simulink model "Test01_SIG_Ctrl_2019a"  (R2019a)
settings: Solver=ode4  StartTime=0.0  StopTime=TMax  FixedStep=DT  MaxStep=DT  RelTol=1e-3  EnableMultiTasking=on
values from neighbouring files (symbols this model uses):
  a0 = -wecs.Bt/wecs.mt    [calcDiscretParamTowerMotion.m]
  a1 = -wecs.Kt/wecs.mt    [calcDiscretParamTowerMotion.m]
  c1 = fmtCell(data{r}(1), nf, doNorm)    [merge_stats_tables_norm.m]
  c2 = fmtCell(data{r}(2), nf, doNorm)    [merge_stats_tables_norm.m]
  IPC_KI_1p = xCtrl(1)    [runSimIPC.m]
  IPC_KP_1p = xCtrl(2)    [runSimIPC.m]
  kp_Turm = xCtrl(3)    [runSimIPC.m]
  OutList = OutTable.Properties.VariableNames    [initLPVParam.m]    (also in testCtrl.m; testOutList.m = cell(40, 1); testqLPV.m = cell(40, 1))
undefined symbols (not defined in the file or in its folder): b0, b0Torque, b1, b1Torque, d1, d2, d3, GBoxEff, GBRatio, GK_Start, IPC_An, IPC_K_1P, k_Pitch, M_Gen_change_max, M_Gen_max, M_Gen_min, MaxPit, MinPit, offest_1p, PC_KI, PC_KK, PC_KP, Pitch_change_max, RPM_Init, strmatch, switchOrigFiltGenSpeed, T_Turmfilter, v_Gen_nenn
libraries: simulink x4, simulink_extras x2
settings Model: Creator=bjonkman  LastModifiedBy=ditt_aj
settings DataIOCC: SaveFormat=Array  SignalLoggingSaveFormat=ModelDataLogs  SaveOutput=off  SaveTime=off  ReturnWorkspaceOutputs=off  SignalLoggingName=sigsOut
settings OptimizationCC: ExpressionDepthLimit=2147483647  LifeSpan=inf
settings DebuggingCC: SaveWithParameterizedLinksMsg=none  UnderspecifiedInitializationDetection=Classic  MergeDetectMultiDrivingBlocksExec=none  SignalResolutionControl=TryResolveAllWithWarning  MultiTaskDSMMsg=warning  MultiTaskCondExecSysMsg=none  FcnCallInpInsideContextMsg=warning  StateNameClashWarn=warning  SFUnexpectedBacktrackingDiag=warning  SFNoUnconditionalDefaultTransitionDiag=warning  ArithmeticOperatorsInVariantConditions=warning
settings HardwareCC: ProdBitPerPointer=32  ProdBitPerSizeT=32  ProdBitPerPtrDiffT=32  ProdLargestAtomicFloat=None  ProdIntDivRoundTo=Undefined  ProdEndianess=Unspecified  ProdWordSize=32  ProdHWDeviceType=32-bit Generic  TargetUnknown=on
settings ModelReferenceCC: PropagateSignalLabelsOutOfModel=off
settings SFSimCC: SimUseLocalCustomCode=off
settings RTWCC: RTWUseLocalCustomCode=off
settings CodeAppCC: StateflowObjectComments=on
settings GRTTargetCC: TargetLangStandard=C89/C90 (ANSI)  ModelReferenceCompliant=off  ParMdlRefBuildCompliant=off  CompOptLevelCompliant=off  ConcurrentExecutionCompliant=off  GeneratePreprocessorConditionals=Disable all  CombineOutputUpdateFcns=off  MatFileLogging=off  GRTInterface=on
settings ConfigComp: CovMetricSettings=dw  CovHtmlReporting=on  CovSaveCumulativeToWorkspaceVar=on  CovSaveSingleToWorkspaceVar=on  CovExternalEMLEnable=off

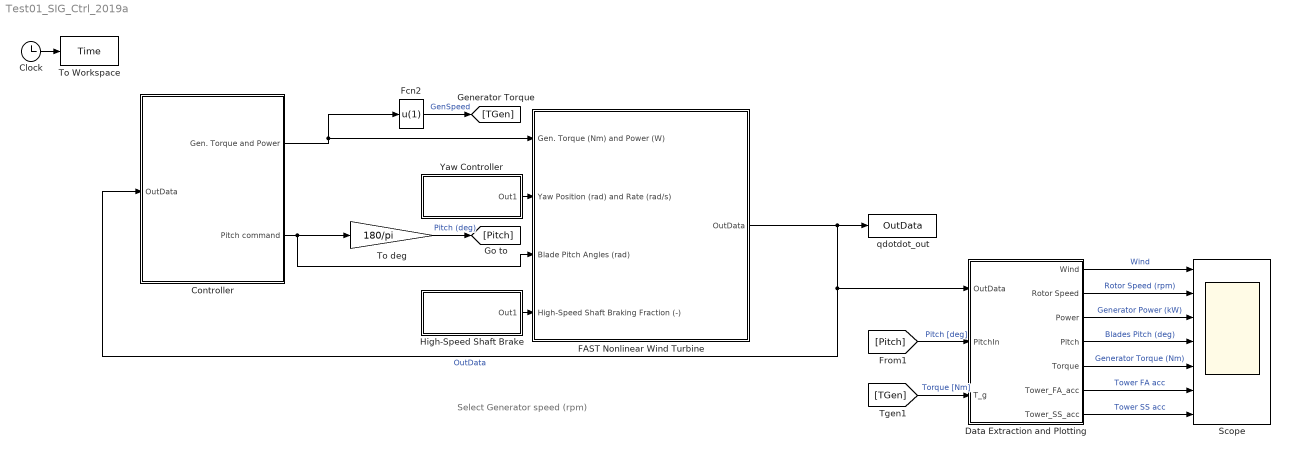
== system Test01_SIG_Ctrl_2019a ==
  note: Select Generator speed (rpm)
  Clock : Clock
  Controller : Subsystem
  Data Extraction and Plotting : Subsystem
  FAST Nonlinear Wind Turbine : Subsystem  mask(FAST Nonlinear Wind Turbine){}
      mask help: This block contains the FAST S-Function.
      mask init:
      | clear FAST_SFunc
  Fcn2 : Fcn  Expr=u(1)
  High-Speed Shaft Brake : Subsystem
  Scope : Scope  NumInputPorts=7
      settings: Tag=Scope
  To Workspace : ToWorkspace  VariableName=Time  SampleTime=-1
  To deg : Gain  Gain=180/pi
  Yaw Controller : Subsystem
  qdotdot_out : ToWorkspace  VariableName=OutData  SampleTime=-1
  wires:
  Clock/1 -> To Workspace/1
  Yaw Controller/1(Out1) -> FAST Nonlinear Wind Turbine/2(Yaw Position (rad) and Rate (rad/s))
  High-Speed Shaft Brake/1(Out1) -> FAST Nonlinear Wind Turbine/4(High-Speed Shaft Braking Fraction (-))
  FAST Nonlinear Wind Turbine/1(OutData) -> qdotdot_out/1, Data Extraction and Plotting/1(OutData), Controller/1(OutData)  "OutData"
  Fcn2/1 -> [TGen]  "GenSpeed"
  Data Extraction and Plotting/2(Rotor Speed) -> Scope/2  "Rotor Speed (rpm)"
  Data Extraction and Plotting/4(Pitch) -> Scope/4  "Blades Pitch (deg)"
  Data Extraction and Plotting/3(Power) -> Scope/3  "Generator Power (kW)"
  [TGen] -> Data Extraction and Plotting/3(T_g)  "Torque [Nm]"
  Data Extraction and Plotting/5(Torque) -> Scope/5  "Generator Torque (Nm)"
  [Pitch] -> Data Extraction and Plotting/2(PitchIn)  "Pitch [deg]"
  Data Extraction and Plotting/7(Tower_SS_acc) -> Scope/7  "Tower SS acc"
  Data Extraction and Plotting/6(Tower_FA_acc) -> Scope/6  "Tower FA acc"
  Data Extraction and Plotting/1(Wind) -> Scope/1  "Wind"
  To deg/1 -> [Pitch]  "Pitch (deg)"
  Controller/2(Pitch command) -> FAST Nonlinear Wind Turbine/3(Blade Pitch Angles (rad)), To deg/1
  Controller/1(Gen. Torque and Power) -> FAST Nonlinear Wind Turbine/1(Gen. Torque (Nm) and Power (W)), Fcn2/1

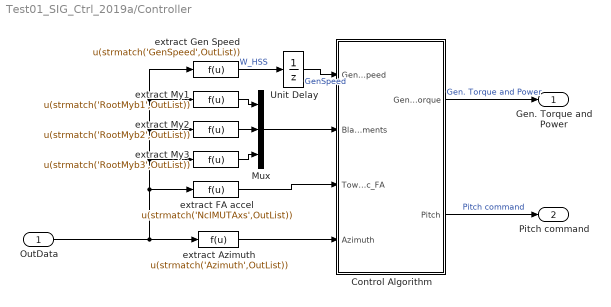
== system Test01_SIG_Ctrl_2019a/Controller ==
  OutData : Inport
  Control Algorithm : Subsystem
  Mux : Mux  Inputs=3
  Unit Delay : UnitDelay  InitialCondition=RPM_Init*GBRatio  SampleTime=-1  HasFrameUpgradeWarning=on
  extract Azimuth : Fcn  Expr=u(strmatch('Azimuth',OutList))
  extract FA accel : Fcn  Expr=u(strmatch('NcIMUTAxs',OutList))
  extract Gen Speed : Fcn  Expr=u(strmatch('GenSpeed',OutList))
  extract My1 : Fcn  Expr=u(strmatch('RootMyb1',OutList))
  extract My2 : Fcn  Expr=u(strmatch('RootMyb2',OutList))
  extract My3 : Fcn  Expr=u(strmatch('RootMyb3',OutList))
  Gen. Torque and Power : Outport
  Pitch command : Outport  Port=2
  wires:
  extract Azimuth/1 -> Control Algorithm/4(Azimuth)
  OutData/1 -> extract Gen Speed/1, extract My1/1, extract My2/1, extract My3/1, extract FA accel/1, extract Azimuth/1
  Unit Delay/1 -> Control Algorithm/1(Generator_Speed)  "GenSpeed"
  extract My3/1 -> Mux/3
  extract FA accel/1 -> Control Algorithm/3(TowerAcc_FA)
  extract My2/1 -> Mux/2
  extract My1/1 -> Mux/1
  Mux/1 -> Control Algorithm/2(Blade_Moments)
  extract Gen Speed/1 -> Unit Delay/1  "W_HSS"
  Control Algorithm/1(Generator_Torque) -> Gen. Torque and Power/1  "Gen. Torque and Power"
  Control Algorithm/2(Pitch) -> Pitch command/1  "Pitch command"

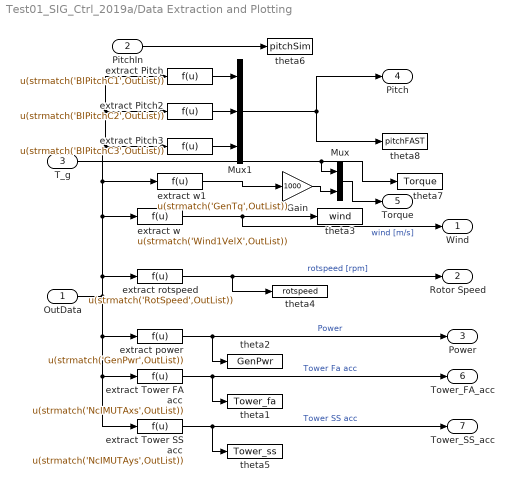
== system Test01_SIG_Ctrl_2019a/Data Extraction and Plotting ==
  OutData : Inport
  PitchIn : Inport  Port=2
  T_g : Inport  Port=3
  Gain : Gain  Gain=1000
  Mux : Mux  Inputs=2
  Mux1 : Mux  Inputs=3
  extract Pitch : Fcn  Expr=u(strmatch('BlPitchC1',OutList))
  extract Pitch2 : Fcn  Expr=u(strmatch('BlPitchC2',OutList))
  extract Pitch3 : Fcn  Expr=u(strmatch('BlPitchC3',OutList))
  extract Tower FA acc : Fcn  Expr=u(strmatch('NcIMUTAxs',OutList))
  extract Tower SS acc : Fcn  Expr=u(strmatch('NcIMUTAys',OutList))
  extract power : Fcn  Expr=u(strmatch('GenPwr',OutList))
  extract rotspeed : Fcn  Expr=u(strmatch('RotSpeed',OutList))
  extract w : Fcn  Expr=u(strmatch('Wind1VelX',OutList))
  extract w1 : Fcn  Expr=u(strmatch('GenTq',OutList))
  theta1 : ToWorkspace  VariableName=Tower_fa  SampleTime=-1
      settings: MaxDataPoints=Inf  Decimation=3
  theta2 : ToWorkspace  VariableName=GenPwr  SampleTime=-1
      settings: MaxDataPoints=Inf  Decimation=3
  theta3 : ToWorkspace  VariableName=wind  SampleTime=-1
      settings: MaxDataPoints=Inf  Decimation=3
  theta4 : ToWorkspace  VariableName=rotspeed  SampleTime=-1
      settings: MaxDataPoints=Inf  Decimation=3
  theta5 : ToWorkspace  VariableName=Tower_ss  SampleTime=-1
      settings: MaxDataPoints=Inf  Decimation=3
  theta6 : ToWorkspace  VariableName=pitchSim  SampleTime=-1
      settings: MaxDataPoints=Inf  Decimation=3
  theta7 : ToWorkspace  VariableName=Torque  SampleTime=-1
      settings: MaxDataPoints=Inf  Decimation=3
  theta8 : ToWorkspace  VariableName=pitchFAST  SampleTime=-1
      settings: MaxDataPoints=Inf  Decimation=3
  Wind : Outport
  Rotor Speed : Outport  Port=2
  Power : Outport  Port=3
  Pitch : Outport  Port=4
  Torque : Outport  Port=5
  Tower_FA_acc : Outport  Port=6
  Tower_SS_acc : Outport  Port=7
  wires:
  extract w/1 -> Wind/1, theta3/1  "wind [m/s]"
  extract rotspeed/1 -> theta4/1, Rotor Speed/1  "rotspeed [rpm]"
  extract power/1 -> theta2/1, Power/1  "Power"
  T_g/1 -> Mux/1, theta7/1
  extract Tower FA acc/1 -> theta1/1, Tower_FA_acc/1  "Tower Fa acc"
  OutData/1 -> extract w/1, extract Pitch/1, extract Pitch2/1, extract Pitch3/1, extract w1/1, extract rotspeed/1, extract Tower SS acc/1, extract Tower FA acc/1, extract power/1
  extract Tower SS acc/1 -> theta5/1, Tower_SS_acc/1  "Tower SS acc"
  extract w1/1 -> Gain/1
  Gain/1 -> Mux/2
  Mux/1 -> Torque/1
  PitchIn/1 -> theta6/1
  Mux1/1 -> theta8/1, Pitch/1
  extract Pitch3/1 -> Mux1/3
  extract Pitch/1 -> Mux1/1
  extract Pitch2/1 -> Mux1/2

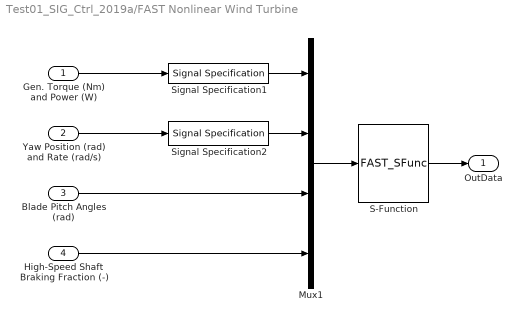
== system Test01_SIG_Ctrl_2019a/FAST Nonlinear Wind Turbine ==
  Gen. Torque (Nm) and Power (W) : Inport
  Yaw Position (rad) and Rate (rad/s) : Inport  Port=2
  Blade Pitch Angles (rad) : Inport  Port=3
  High-Speed Shaft Braking Fraction (-) : Inport  Port=4
  Mux1 : Mux
  S-Function : S-Function  FunctionName=FAST_SFunc  Parameters=FAST_InputFileName, TMax, 0  SFunctionDeploymentMode=off  EnableBusSupport=off
  Signal Specification1 : SignalSpecification  OutDataTypeStr=double  Dimensions=2
  Signal Specification2 : SignalSpecification  OutDataTypeStr=double  Dimensions=2
  OutData : Outport
  wires:
  Gen. Torque (Nm) and Power (W)/1 -> Signal Specification1/1
  S-Function/1 -> OutData/1
  Mux1/1 -> S-Function/1
  Blade Pitch Angles (rad)/1 -> Mux1/3
  Yaw Position (rad) and Rate (rad/s)/1 -> Signal Specification2/1
  Signal Specification1/1 -> Mux1/1
  Signal Specification2/1 -> Mux1/2
  High-Speed Shaft Braking Fraction (-)/1 -> Mux1/4

== system Test01_SIG_Ctrl_2019a/High-Speed Shaft Brake ==
  High-Speed Shaft Braking Fraction : Constant  Value=0
  Out1 : Outport
  wires:
  High-Speed Shaft Braking Fraction/1 -> Out1/1

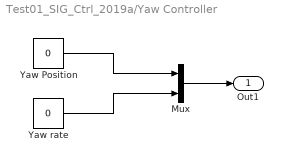
== system Test01_SIG_Ctrl_2019a/Yaw Controller ==
  Mux : Mux  Inputs=2
  Yaw Position : Constant  Value=0
  Yaw rate : Constant  Value=0
  Out1 : Outport
  wires:
  Mux/1 -> Out1/1
  Yaw Position/1 -> Mux/1
  Yaw rate/1 -> Mux/2

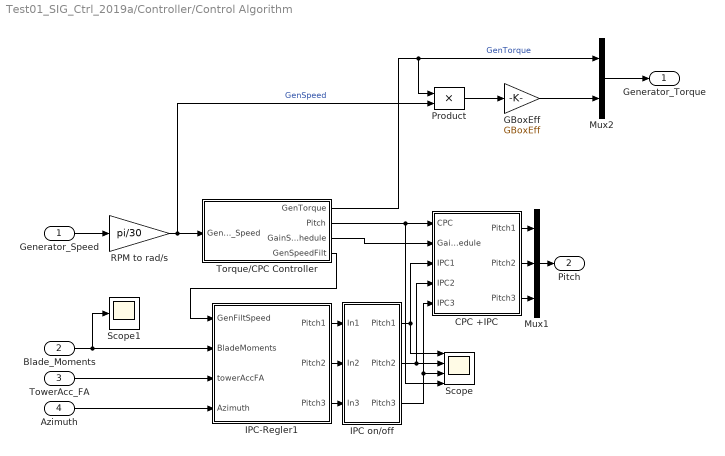
== system Test01_SIG_Ctrl_2019a/Controller/Control Algorithm ==
  Generator_Speed : Inport
  Blade_Moments : Inport  Port=2
  TowerAcc_FA : Inport  Port=3
  Azimuth : Inport  Port=4
  CPC +IPC : Subsystem
  GBoxEff : Gain  Gain=GBoxEff
  IPC on/off : Subsystem
  IPC-Regler1 : Subsystem
  Mux1 : Mux  Inputs=3
  Mux2 : Mux  Inputs=2
  Product : Product  RndMeth=Zero
  RPM to rad/s : Gain  Gain=pi/30  SaturateOnIntegerOverflow=on  OutDataTypeStr=Inherit: Same as input  ParamDataTypeStr=Inherit: Same as input
  Scope : Scope  NumInputPorts=4
  Scope1 : Scope
  Torque/CPC Controller : Subsystem
  Generator_Torque : Outport
  Pitch : Outport  Port=2
  wires:
  IPC on/off/3(Pitch3) -> CPC +IPC/5(IPC3), Scope/3
  Torque/CPC Controller/4(GenSpeedFilt) -> IPC-Regler1/1(GenFiltSpeed)
  IPC on/off/1(Pitch1) -> CPC +IPC/3(IPC1), Scope/1
  Torque/CPC Controller/2(Pitch) -> Scope/4, CPC +IPC/1(CPC)
  CPC +IPC/3(Pitch3) -> Mux1/3
  IPC on/off/2(Pitch2) -> CPC +IPC/4(IPC2), Scope/2
  IPC-Regler1/3(Pitch3) -> IPC on/off/3(In3)
  IPC-Regler1/1(Pitch1) -> IPC on/off/1(In1)
  IPC-Regler1/2(Pitch2) -> IPC on/off/2(In2)
  Torque/CPC Controller/3(GainSchedule) -> CPC +IPC/2(GainSchedule)
  CPC +IPC/1(Pitch1) -> Mux1/1
  CPC +IPC/2(Pitch2) -> Mux1/2
  Azimuth/1 -> IPC-Regler1/4(Azimuth)
  Torque/CPC Controller/1(GenTorque) -> Mux2/1, Product/1  "GenTorque"
  Blade_Moments/1 -> Scope1/1, IPC-Regler1/2(BladeMoments)
  Mux1/1 -> Pitch/1
  TowerAcc_FA/1 -> IPC-Regler1/3(towerAccFA)
  Product/1 -> GBoxEff/1
  Generator_Speed/1 -> RPM to rad/s/1
  GBoxEff/1 -> Mux2/2
  Mux2/1 -> Generator_Torque/1
  RPM to rad/s/1 -> Product/2, Torque/CPC Controller/1(Generator_Speed)  "GenSpeed"

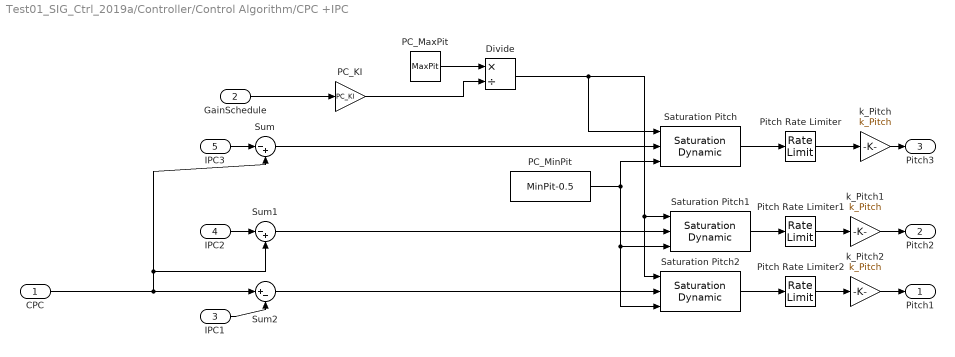
== system Test01_SIG_Ctrl_2019a/Controller/Control Algorithm/CPC +IPC ==
  CPC : Inport
  GainSchedule : Inport  Port=2
  IPC1 : Inport  Port=3
  IPC2 : Inport  Port=4
  IPC3 : Inport  Port=5
  Divide : Product  Inputs=*/
  PC_KI : Gain  Gain=PC_KI
  PC_MaxPit : Constant  Value=MaxPit
  PC_MinPit : Constant  Value=MinPit-0.5
  Pitch Rate Limiter : RateLimiter  RisingSlewLimit=Pitch_change_max  FallingSlewLimit=-Pitch_change_max  SampleTimeMode=inherited
  Pitch Rate Limiter1 : RateLimiter  RisingSlewLimit=Pitch_change_max  FallingSlewLimit=-Pitch_change_max  SampleTimeMode=inherited
  Pitch Rate Limiter2 : RateLimiter  RisingSlewLimit=Pitch_change_max  FallingSlewLimit=-Pitch_change_max  SampleTimeMode=inherited
  Saturation Pitch : simulink/Discontinuities/Saturation Dynamic  OutMin=[]  OutMax=[]  OutDataTypeStr=Inherit: Same as second input  OutDataType=fixdt(1, 16)  OutScaling=2^-10  DoSatur=off
  Saturation Pitch1 : simulink/Discontinuities/Saturation Dynamic  OutMin=[]  OutMax=[]  OutDataTypeStr=Inherit: Same as second input  OutDataType=fixdt(1, 16)  OutScaling=2^-10  DoSatur=off
  Saturation Pitch2 : simulink/Discontinuities/Saturation Dynamic  OutMin=[]  OutMax=[]  OutDataTypeStr=Inherit: Same as second input  OutDataType=fixdt(1, 16)  OutScaling=2^-10  DoSatur=off
  Sum : Sum  Inputs=|-+
  Sum1 : Sum  Inputs=|-+
  Sum2 : Sum  Inputs=|+-
  k_Pitch : Gain  Gain=k_Pitch
  k_Pitch1 : Gain  Gain=k_Pitch
  k_Pitch2 : Gain  Gain=k_Pitch
  Pitch1 : Outport
  Pitch2 : Outport  Port=2
  Pitch3 : Outport  Port=3
  wires:
  PC_KI/1 -> Divide/2
  PC_MinPit/1 -> Saturation Pitch1/3, Saturation Pitch2/3, Saturation Pitch/3
  Saturation Pitch/1 -> Pitch Rate Limiter/1
  Pitch Rate Limiter1/1 -> k_Pitch1/1
  Divide/1 -> Saturation Pitch1/1, Saturation Pitch2/1, Saturation Pitch/1
  Pitch Rate Limiter2/1 -> k_Pitch2/1
  Pitch Rate Limiter/1 -> k_Pitch/1
  Sum1/1 -> Saturation Pitch1/2
  PC_MaxPit/1 -> Divide/1
  Sum2/1 -> Saturation Pitch2/2
  IPC3/1 -> Sum/1
  Saturation Pitch1/1 -> Pitch Rate Limiter1/1
  k_Pitch1/1 -> Pitch2/1
  Sum/1 -> Saturation Pitch/2
  Saturation Pitch2/1 -> Pitch Rate Limiter2/1
  IPC2/1 -> Sum1/1
  k_Pitch/1 -> Pitch3/1
  GainSchedule/1 -> PC_KI/1
  IPC1/1 -> Sum2/2
  CPC/1 -> Sum1/2, Sum/2, Sum2/1
  k_Pitch2/1 -> Pitch1/1

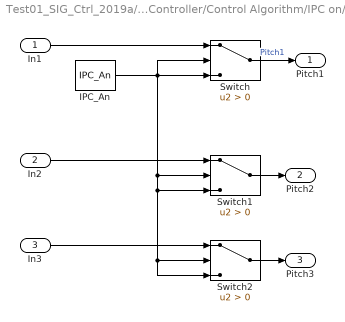
== system Test01_SIG_Ctrl_2019a/Controller/Control Algorithm/IPC on//off ==
  In1 : Inport
  In2 : Inport  Port=2
  In3 : Inport  Port=3
  IPC_An : Constant  Value=IPC_An
  Switch : Switch  Criteria=u2 > Threshold
  Switch1 : Switch  Criteria=u2 > Threshold
  Switch2 : Switch  Criteria=u2 > Threshold
  Pitch1 : Outport
  Pitch2 : Outport  Port=2
  Pitch3 : Outport  Port=3
  wires:
  Switch1/1 -> Pitch2/1
  IPC_An/1 -> Switch1/2, Switch1/3, Switch2/2, Switch2/3, Switch/3, Switch/2
  In3/1 -> Switch2/1
  In1/1 -> Switch/1
  In2/1 -> Switch1/1
  Switch/1 -> Pitch1/1  "Pitch1"
  Switch2/1 -> Pitch3/1

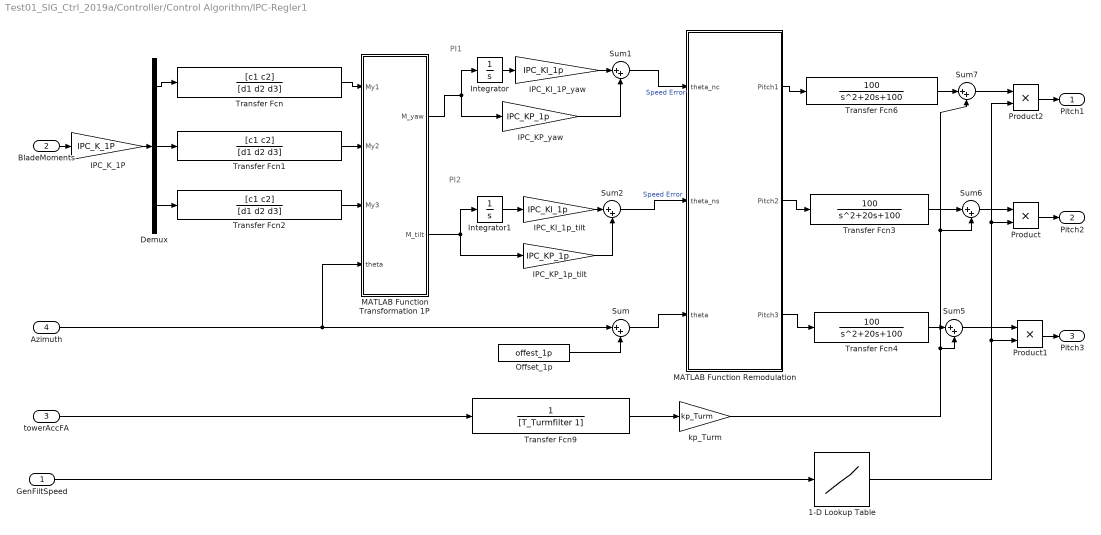
== system Test01_SIG_Ctrl_2019a/Controller/Control Algorithm/IPC-Regler1 ==
  note: PI2
  note: PI1
  GenFiltSpeed : Inport
  BladeMoments : Inport  Port=2
  towerAccFA : Inport  Port=3
  Azimuth : Inport  Port=4
  1-D Lookup Table : Lookup_n-D  NumberOfTableDimensions=1  BreakpointsForDimension1=[0 0.8*v_Gen_nenn 0.9*v_Gen_nenn 1000]  Table=[0 0 1 1]  InternalRulePriority=Speed  RndMeth=Simplest  InputSameDT=on
  Demux : Demux  Outputs=3
  IPC_KI_1P_yaw : Gain  Gain=IPC_KI_1p
  IPC_KI_1p_tilt : Gain  Gain=IPC_KI_1p
  IPC_KP_1p_tilt : Gain  Gain=IPC_KP_1p
  IPC_KP_yaw : Gain  Gain=IPC_KP_1p
  IPC_K_1P : Gain  Gain=IPC_K_1P
  Integrator : Integrator
  Integrator1 : Integrator  LimitOutput=on  UpperSaturationLimit=90  LowerSaturationLimit=-90
  MATLAB Function Remodulation : MATLAB Function  TreatAsAtomicUnit=on
  MATLAB Function Transformation 1P : MATLAB Function  TreatAsAtomicUnit=on
  Offset_1p : Constant  Value=offest_1p
  Product : Product
  Product1 : Product
  Product2 : Product
  Sum{,1..2,5..7} (6 alike) : Sum  Inputs=|++
  Transfer Fcn : TransferFcn  Numerator=[c1 c2]  Denominator=[d1 d2 d3]
  Transfer Fcn1 : TransferFcn  Numerator=[c1 c2]  Denominator=[d1 d2 d3]
  Transfer Fcn2 : TransferFcn  Numerator=[c1 c2]  Denominator=[d1 d2 d3]
  Transfer Fcn3 : TransferFcn  Numerator=100  Denominator=[1 20 100]
  Transfer Fcn4 : TransferFcn  Numerator=100  Denominator=[1 20 100]
  Transfer Fcn6 : TransferFcn  Numerator=100  Denominator=[1 20 100]
  Transfer Fcn9 : TransferFcn  Numerator=1  Denominator=[T_Turmfilter 1]
  kp_Turm : Gain  Gain=kp_Turm
  Pitch1 : Outport
  Pitch2 : Outport  Port=2
  Pitch3 : Outport  Port=3
  wires:
  Azimuth/1 -> MATLAB Function Transformation 1P/4(theta), Sum/1
  kp_Turm/1 -> Sum6/2, Sum7/2, Sum5/2
  Transfer Fcn9/1 -> kp_Turm/1
  Sum5/1 -> Product1/1
  Product2/1 -> Pitch1/1
  1-D Lookup Table/1 -> Product1/2, Product/2, Product2/2
  Product1/1 -> Pitch3/1
  Product/1 -> Pitch2/1
  Sum6/1 -> Product/1
  Sum7/1 -> Product2/1
  GenFiltSpeed/1 -> 1-D Lookup Table/1
  towerAccFA/1 -> Transfer Fcn9/1
  Transfer Fcn6/1 -> Sum7/1
  Transfer Fcn3/1 -> Sum6/1
  Transfer Fcn4/1 -> Sum5/1
  MATLAB Function Remodulation/3(Pitch3) -> Transfer Fcn4/1
  MATLAB Function Remodulation/2(Pitch2) -> Transfer Fcn3/1
  MATLAB Function Remodulation/1(Pitch1) -> Transfer Fcn6/1
  Offset_1p/1 -> Sum/2
  Sum/1 -> MATLAB Function Remodulation/3(theta)
  IPC_K_1P/1 -> Demux/1
  Transfer Fcn2/1 -> MATLAB Function Transformation 1P/3(My3)
  Transfer Fcn/1 -> MATLAB Function Transformation 1P/1(My1)
  Transfer Fcn1/1 -> MATLAB Function Transformation 1P/2(My2)
  BladeMoments/1 -> IPC_K_1P/1
  Demux/3 -> Transfer Fcn2/1
  Demux/2 -> Transfer Fcn1/1
  Demux/1 -> Transfer Fcn/1
  IPC_KI_1P_yaw/1 -> Sum1/1
  IPC_KP_yaw/1 -> Sum1/2
  Integrator/1 -> IPC_KI_1P_yaw/1
  Sum1/1 -> MATLAB Function Remodulation/1(theta_nc)  "Speed Error"
  MATLAB Function Transformation 1P/1(M_yaw) -> Integrator/1, IPC_KP_yaw/1
  Sum2/1 -> MATLAB Function Remodulation/2(theta_ns)  "Speed Error"
  Integrator1/1 -> IPC_KI_1p_tilt/1
  IPC_KP_1p_tilt/1 -> Sum2/2
  IPC_KI_1p_tilt/1 -> Sum2/1
  MATLAB Function Transformation 1P/2(M_tilt) -> Integrator1/1, IPC_KP_1p_tilt/1

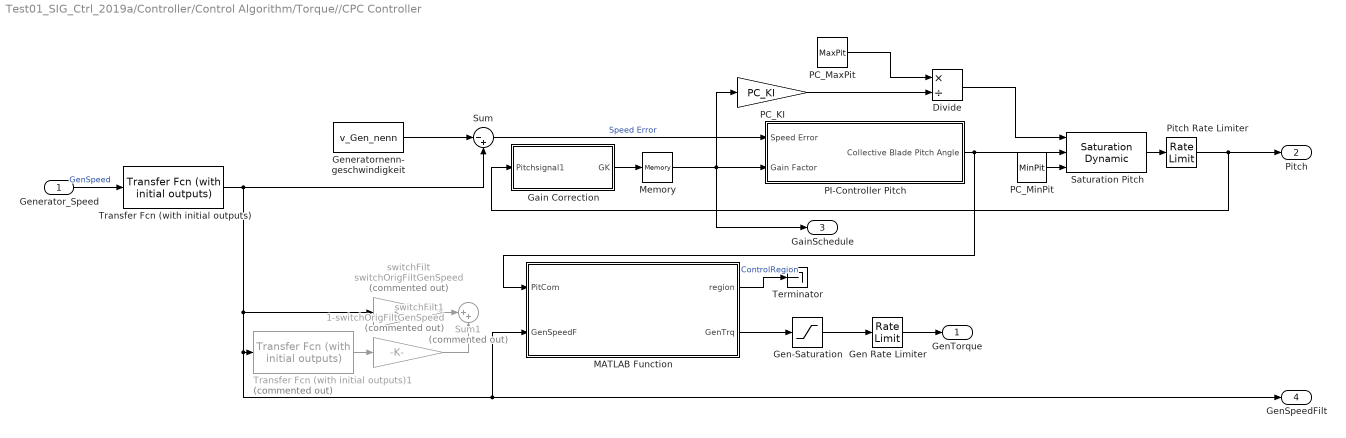
== system Test01_SIG_Ctrl_2019a/Controller/Control Algorithm/Torque//CPC Controller ==
  Generator_Speed : Inport
  Divide : Product  Inputs=*/
  Gain Correction : Subsystem
  Gen Rate Limiter : RateLimiter  RisingSlewLimit=M_Gen_change_max  FallingSlewLimit=-M_Gen_change_max
  Gen-Saturation : Saturate  UpperLimit=M_Gen_max  LowerLimit=M_Gen_min
  Generatornenn- geschwindigkeit : Constant  Value=v_Gen_nenn
  MATLAB Function : MATLAB Function  TreatAsAtomicUnit=on
  Memory : Memory  InitialCondition=1  InheritSampleTime=on
  PC_KI : Gain  Gain=PC_KI
  PC_MaxPit : Constant  Value=MaxPit
  PC_MinPit : Constant  Value=MinPit
  PI-Controller Pitch : Subsystem
  Pitch Rate Limiter : RateLimiter  RisingSlewLimit=Pitch_change_max  FallingSlewLimit=-Pitch_change_max  SampleTimeMode=inherited
  Saturation Pitch : simulink/Discontinuities/Saturation Dynamic  OutMin=[]  OutMax=[]  OutDataTypeStr=Inherit: Same as second input  OutDataType=fixdt(1, 16)  OutScaling=2^-10  DoSatur=off
  Sum : Sum  Inputs=|-+
  Sum1 : Sum  Commented=on  Inputs=|++
  Terminator : Terminator
  Transfer Fcn (with initial outputs) : simulink_extras/Additional Linear/Transfer Fcn (with initial outputs)  N=[a1 a0]  D=[b1 b0]  Y0=RPM_Init*GBRatio *pi/30  U0=RPM_Init*GBRatio *pi/30
  Transfer Fcn (with initial outputs)1 : simulink_extras/Additional Linear/Transfer Fcn (with initial outputs)  Commented=on  N=1  D=[b1Torque*5 b0Torque]  Y0=RPM_Init*GBRatio *pi/30  U0=RPM_Init*GBRatio *pi/30
  switchFilt : Gain  Commented=on  Gain=switchOrigFiltGenSpeed
  switchFilt1 : Gain  Commented=on  Gain=1-switchOrigFiltGenSpeed
  GenTorque : Outport
  Pitch : Outport  Port=2
  GainSchedule : Outport  Port=3
  GenSpeedFilt : Outport  Port=4
  wires:
  Sum/1 -> PI-Controller Pitch/1(Speed Error)  "Speed Error"
  PI-Controller Pitch/1(Collective Blade Pitch Angle) -> Saturation Pitch/2, MATLAB Function/1(PitCom)
  Gen Rate Limiter/1 -> GenTorque/1
  Saturation Pitch/1 -> Pitch Rate Limiter/1
  PC_MinPit/1 -> Saturation Pitch/3
  PC_KI/1 -> Divide/2
  PC_MaxPit/1 -> Divide/1
  Divide/1 -> Saturation Pitch/1
  Gen-Saturation/1 -> Gen Rate Limiter/1
  Generatornenn- geschwindigkeit/1 -> Sum/1
  MATLAB Function/2(GenTrq) -> Gen-Saturation/1
  Transfer Fcn (with initial outputs)/1 -> Sum/2, switchFilt/1, Transfer Fcn (with initial outputs)1/1, MATLAB Function/2(GenSpeedF), GenSpeedFilt/1
  MATLAB Function/1(region) -> Terminator/1  "ControlRegion"
  Pitch Rate Limiter/1 -> Gain Correction/1(Pitchsignal1), Pitch/1
  Gain Correction/1(GK) -> Memory/1
  Generator_Speed/1 -> Transfer Fcn (with initial outputs)/1  "GenSpeed"
  Memory/1 -> PI-Controller Pitch/2(Gain Factor), GainSchedule/1, PC_KI/1
  Transfer Fcn (with initial outputs)1/1 -> switchFilt1/1
  switchFilt/1 -> Sum1/1
  switchFilt1/1 -> Sum1/2

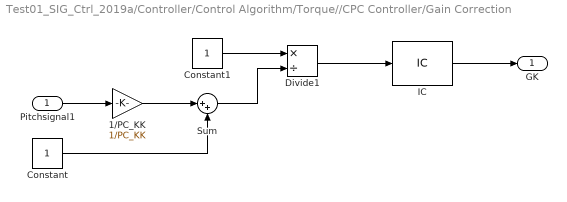
== system Test01_SIG_Ctrl_2019a/Controller/Control Algorithm/Torque//CPC Controller/Gain Correction ==
  Pitchsignal1 : Inport
  1/PC_KK : Gain  Gain=1/PC_KK
  Constant : Constant
  Constant1 : Constant
  Divide1 : Product  Inputs=*/
  IC : InitialCondition  Value=GK_Start
  Sum : Sum  Inputs=|++
  GK : Outport
  wires:
  Pitchsignal1/1 -> 1/PC_KK/1
  Constant/1 -> Sum/2
  Constant1/1 -> Divide1/1
  Sum/1 -> Divide1/2
  1/PC_KK/1 -> Sum/1
  Divide1/1 -> IC/1
  IC/1 -> GK/1

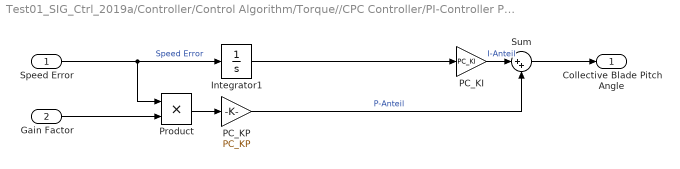
== system Test01_SIG_Ctrl_2019a/Controller/Control Algorithm/Torque//CPC Controller/PI-Controller Pitch ==
  Speed Error : Inport
  Gain Factor : Inport  Port=2
  Integrator1 : Integrator  LimitOutput=on  UpperSaturationLimit=90  LowerSaturationLimit=0
  PC_KI : Gain  Gain=PC_KI
  PC_KP : Gain  Gain=PC_KP
  Product : Product
  Sum : Sum  Inputs=|++
  Collective Blade Pitch Angle : Outport
  wires:
  Speed Error/1 -> Integrator1/1, Product/1  "Speed Error"
  Sum/1 -> Collective Blade Pitch Angle/1
  PC_KI/1 -> Sum/1  "I-Anteil"
  PC_KP/1 -> Sum/2  "P-Anteil"
  Product/1 -> PC_KP/1
  Gain Factor/1 -> Product/2
  Integrator1/1 -> PC_KI/1

== matlab function Test01_SIG_Ctrl_2019a/Controller/Control Algorithm/Torque//CPC Controller/MATLAB Function ==
  data: PitCom input; region output; GenSpeedF input; GenTrq output
function [region,GenTrq] = fcn(PitCom,GenSpeedF)
%#codegen

if GenSpeedF >= 121.6805  % | (  PitCom(1) >= 0.01745329) ) % We are in region 3 - power is constant
         GenTrq =  5296610/GenSpeedF; %4.3094e+04; %
         region=3;
%          if  GenSpeedF>=125
%              GenTrq =721/5*GenSpeedF+24348; %2648305*GenSpeedF + 2.1187e+04; %-18.0834*GenSpeedF+4.3094e+04;
%          end
%          if GenSpeedF>=130
%              GenTrq =4.3094e+04;
%          end

elseif ( GenSpeedF <= 70.16224 )           % We are in region 1 - torque is zero
         GenTrq = 0.0;
         region=1;
elseif ( GenSpeedF <  91.21091 ) % We are in region 1 1/2 - linear ramp in torque from zero to optimal
         GenTrq = 921.83015253225492464369482727412*( GenSpeedF - 70.16224);
         region = 1.5;
elseif ( GenSpeedF <  119.0138 )  % We are in region 2 - optimal torque is proportional to the square of the generator speed
         GenTrq = 2.332287*GenSpeedF*GenSpeedF;
         region = 2;
else                                           % We are in region 2 1/2 - simple induction generator transition region
         GenTrq = 3.9350e+03*( GenSpeedF - 110.6186);
         region = 2.5;
end

== matlab function Test01_SIG_Ctrl_2019a/Controller/Control Algorithm/IPC-Regler1/MATLAB Function Remodulation ==
  data: theta_nc input; Pitch1 output; theta_ns input; Pitch2 output; Pitch3 output; theta input
function [Pitch1,Pitch2,Pitch3] = remodulation(theta_nc,theta_ns,theta)
%#codegen
Pitch=[cos(theta)          sin(theta);...
       cos(theta+2*pi/3) sin(theta+2*pi/3);...
       cos(theta+4*pi/3) sin(theta+4*pi/3)] *[theta_nc;theta_ns];
   
   Pitch1 = Pitch(1);
   Pitch2 = Pitch(2);
   Pitch3 = Pitch(3);

== matlab function Test01_SIG_Ctrl_2019a/Controller/Control Algorithm/IPC-Regler1/MATLAB Function Transformation 1P ==
  data: My1 input; M_yaw output; My2 input; My3 input; M_tilt output; theta input
function [M_yaw,M_tilt] = demodulation(My1,My2,My3,theta)
% Coleman Transformation: D-q transformation of blade moments
% https://en.wikipedia.org/wiki/Direct%E2%80%93quadrature%E2%80%93zero_transformation
% 
% Inputs
%  - Blade root moments in rotating frame: My1,My2,My3
%  - Azimuth
% Outputs 
%  - M_Yaw: Mnc, moment around tower, Axis positiv upwards
%  - M_tilt: Mns, quadrature-axis (um y (Achse weder in Windrichtung  noch nach oben))

%#codegen
Mout=[cos(theta) cos((theta+2*pi/3)) cos((theta+4*pi/3));...
      sin(theta) sin((theta+2*pi/3)) sin((theta+4*pi/3))] *[My1;My2;My3];

M_yaw  = 2/3*Mout(1);
M_tilt = 2/3*Mout(2);
